simulink model "Temperture"  (R2013a)
settings: Solver=ode45  StartTime=0.0  StopTime=10  RelTol=1e-3
values from neighbouring files (symbols this model uses):
  Q1 = (hi*Ai+minf*Cp+Msupply*Cp)/(m*Cp)    (= 4.53572335601)    [EE.m]
undefined symbols (not defined in the file or in its folder): Q2
settings Model: Creator=Mojtaba  LastModifiedBy=Mojtaba

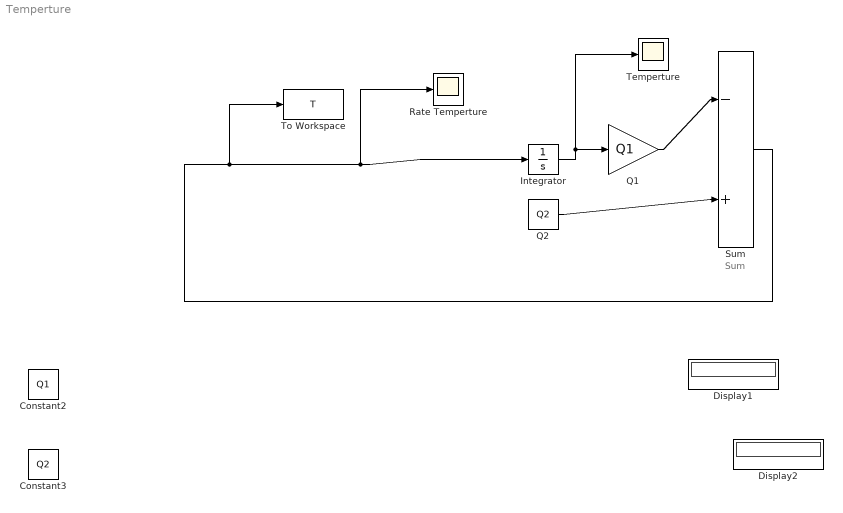
== system Temperture ==
  note: Sum
  Constant2 : Constant  Value=Q1
  Constant3 : Constant  Value=Q2
  Display1 : Display
  Display2 : Display
  Integrator : Integrator  InitialCondition=10
  Q1 : Gain  Gain=Q1
  Q2 : Constant  Value=Q2
  "Rate Temperture " : Scope
  Sum : Sum  Inputs=|-+
  Temperture : Scope
      settings: SaveName=ScopeData2
  To Workspace : ToWorkspace  VariableName=T  SampleTime=-1  SaveFormat=Structure With Time
  wires:
  Integrator/1 -> Temperture/1, Q1/1
  Q1/1 -> Sum/1
  Q2/1 -> Sum/2
  Sum/1 -> Integrator/1, "Rate Temperture "/1, To Workspace/1
